simulink model "danxiangquanqiaozhengliudianlu_R"  (R2025a)
settings: Solver=ode23tb  StartTime=0.0  StopTime=1  MaxStep=1e-5  RelTol=1e-5
libraries: spsThyristorLib x4, spsACVoltageSourceLib x1, spsMultimeterLib x1, spsSeriesRLCBranchLib x1, sps_lib x1
settings Model: Creator=小鱼  LastModifiedBy=小鱼

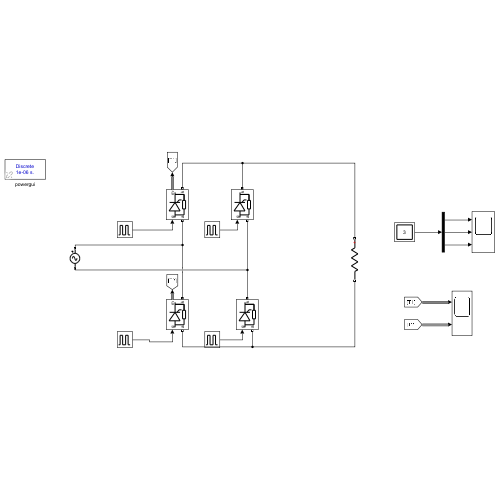
[thumbnail: Simulink's stored preview of the top-level diagram]
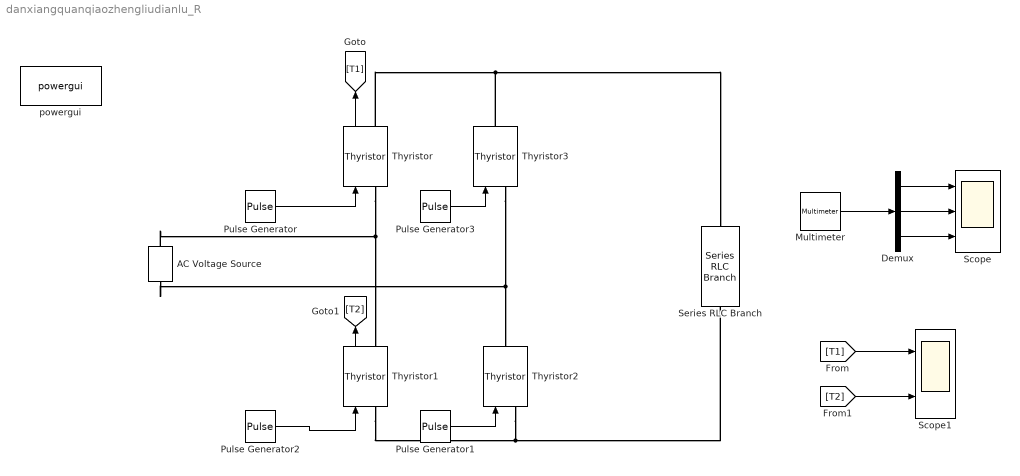
== system danxiangquanqiaozhengliudianlu_R ==
  AC Voltage Source : spsACVoltageSourceLib/AC Voltage Source  Amplitude=220*sqrt(2)  Phase=0  Frequency=50  SampleTime=-1  Measurements=Voltage  BusType=swing  Pref=10e3  Qref=0  Qmin=-inf  Qmax=+inf
  Demux : Demux  Outputs=3
  Multimeter : spsMultimeterLib/Multimeter  L=3  sel=[2 1 3]  yselected={}  Gain=[1 1 1]  OutputType=Complex  PlotAtSimulationStop=off  PhasorSimulation=off
  Pulse Generator : DiscretePulseGenerator  PulseType=Time based  Period=0.02  PulseWidth=5  PhaseDelay=45/360*0.02
  Pulse Generator1 : DiscretePulseGenerator  PulseType=Time based  Period=0.02  PulseWidth=5  PhaseDelay=45/360*0.02
  Pulse Generator2 : DiscretePulseGenerator  PulseType=Time based  Period=0.02  PulseWidth=5  PhaseDelay=(45+180)/360*0.02
  Pulse Generator3 : DiscretePulseGenerator  PulseType=Time based  Period=0.02  PulseWidth=5  PhaseDelay=45/360*0.02
  Scope : Scope  NumInputPorts=3
      settings: ActiveDisplayYMinimum=-388.90872966867204  ActiveDisplayYMaximum=388.9087296685417
  Scope1 : Scope  NumInputPorts=2
      settings: ActiveDisplayYMinimum=-128.95493697814209  ActiveDisplayYMaximum=339.34350501881505
  Series RLC Branch : spsSeriesRLCBranchLib/Series RLC Branch  LConnTagsString=__new0  RConnTagsString=__new0  BranchType=R  Resistance=10  Inductance=1e-3  SetiL0=off  InitialCurrent=0  Capacitance=1e-6  Setx0=off  InitialVoltage=0  Measurements=Branch voltage and current
  Thyristor : spsThyristorLib/Thyristor  Ron=0.001  Lon=0  Vf=0.8  IC=0  Rs=500  Cs=250e-9  Measurements=on
  Thyristor1 : spsThyristorLib/Thyristor  Ron=0.001  Lon=0  Vf=0.8  IC=0  Rs=500  Cs=250e-9  Measurements=on
  Thyristor2 : spsThyristorLib/Thyristor  Ron=0.001  Lon=0  Vf=0.8  IC=0  Rs=500  Cs=250e-9  Measurements=off
  Thyristor3 : spsThyristorLib/Thyristor  Ron=0.001  Lon=0  Vf=0.8  IC=0  Rs=500  Cs=250e-9  Measurements=off
  powergui : sps_lib/powergui  Priority=1  SimulationMode=Discrete  SampleTime=1e-6  frequency=60  Iterations=50  frequencyindice=50  Pbase=100e6  ErrMax=1e-4  UnitsV=kV  UnitsW=MW  buscounter=0  FunctionMessages=off  echomessages=off  EnableUseOfTLC=off  CurrentSourceSwitches=off  DisableSnubberDevices=off  DisableRonSwitches=off  DisableVfSwitches=off  DisplayEquations=off  AutomaticDiscreteSolvers=off  SolverType=Tustin/Backward Euler (TBE)  Interpol=off  ExternalGateDelay=off  methode=off  Ts=100  x0status=blocks  SPID=on  SwTol=0  HookPort=off  NonlinearTolerance=1e-4  nMaxIteration=100  ContinueOnMaxIteration=off  RestoreLinks=warning  ResistiveCurrentMeasurement=off  Frange=[0:2:500]  Ylog=off  Xlog=on  ShowGrid=off  save=off  variable=ZData  structure=0  ZoomFFT=off  StartTime=0.0  cycles=1  DisplayStyle=1  fundamental=60  FreqAxis=off  MaxFrequency=1000  frequencyindicesteady=1  RmsSteady=1  display=off
  wires:
  Pulse Generator/1 -> Thyristor/1
  Pulse Generator1/1 -> Thyristor2/1
  Pulse Generator2/1 -> Thyristor1/1
  Pulse Generator3/1 -> Thyristor3/1
  Multimeter/1 -> Demux/1
  Demux/2 -> Scope/2
  Demux/1 -> Scope/1
  Demux/3 -> Scope/3
  Thyristor/1 -> [T1]
  Thyristor1/1 -> [T2]
  [T1] -> Scope1/1
  [T2] -> Scope1/2
  connections:
  Thyristor/LConn1 -- AC Voltage Source/RConn1 -- Thyristor1/RConn1
  Thyristor3/LConn1 -- AC Voltage Source/LConn1 -- Thyristor2/RConn1
  Thyristor/RConn1 -- Series RLC Branch/LConn1 -- Thyristor3/RConn1
  Thyristor1/LConn1 -- Series RLC Branch/RConn1 -- Thyristor2/LConn1
